simulink model "infinity_mobile_manipulator"  (R2025b)
settings: Solver=ode23t  StartTime=0.0  StopTime=30.0  MaxStep=0.01  RelTol=1e-3  AbsTol=1e-3  EnableMultiTasking=on
undefined symbols (not defined in the file): A, armP, goal, lemP, qa, qb, qHome, Ta, X, Y, Z
libraries: sm_lib x60, nesl_utility x12
(part 2 of 2)

== matlab function infinity_mobile_manipulator/gate ==
  data: v input; w input; vo output; phase input; wo output
function [vo, wo] = gate(v, w, phase)
% Drive only during Navigate/Settle (phase 0); stand still afterwards
if phase == 0
    vo = v; wo = w;
else
    vo = 0; wo = 0;
end

== matlab function infinity_mobile_manipulator/go to goal ==
  data: x input; y input; v output; th input; goal input; w output; reached output
function [v, w, reached] = goToGoal(x, y, th, goal)
kv = 0.6; kw = 2.0; tol = 0.03; vmax = 0.7; wmax = 1.5;   % vmax = QBot nominal speed
dx = goal(1) - x;  dy = goal(2) - y;
rho   = hypot(dx, dy);
ang   = atan2(dy, dx);
alpha = atan2(sin(ang - th), cos(ang - th));              % heading error, wrapped
reached = rho < tol;
if reached
    v = 0; w = 0;
else
    v = min(kv*rho*max(cos(alpha), 0), vmax);
    w = max(min(kw*alpha, wmax), -wmax);
end
end

== stateflow chart infinity_mobile_manipulator/Superviser ==
  settings: updateMethod=DISCRETE  sampleTime=0.01
  state Navigate
    entry:
    phase=0;
    tEnter = tClk;
  state Settle
    entry:
    phase = 0;
    tEnter = tClk;
  state Approach
    entry:
    phase = 1;
    tEnter = tClk;
  state Trace
    entry:
    phase = 2;
    tEnter = tClk;
  (default) -> Navigate
  Navigate -> Settle : [reached]
  Settle -> Approach : [tClk - tEnter >= 1]
  Approach -> Trace : [tClk - tEnter >= 4]
  data: tEnter output double; reached input; phase output double; tClk input double

== matlab function infinity_mobile_manipulator/armRef ==
  data: phase input; qref output; t input; tEnter input; armP input; lemP input; qHome input; Ta input; pd output
function [qref, pd] = armRef(phase, t, tEnter, armP, lemP, qHome, Ta)
qh = qHome(:);
tp = max(t - tEnter, 0);
pStart = lemniscate(0, lemP);
if phase == 1                               % Approach: stowed -> start of the infinity
    u = min(tp/Ta, 1);  s = 3*u^2 - 2*u^3;  % smoothstep
    qref = (1-s)*qh + s*ik4(pStart, armP);
    pd = pStart;
elseif phase == 2                           % Trace: repeats forever
    pd = lemniscate(tp, lemP);
    qref = ik4(pd, armP);
else                                        % Navigate / Settle: stowed
    qref = qh;  pd = pStart;
end
end

function p = lemniscate(t, P)               % P = [cx cy a z w]
d = 1 + sin(P(5)*t)^2;
p = [P(1) + P(3)*cos(P(5)*t)/d;
     P(2) + P(3)*sin(P(5)*t)*cos(P(5)*t)/d;
     P(4)];
end

function q = ik4(p, A)                      % A = [h1 L2 L3 L4], gripper pointing down
h1 = A(1); L2 = A(2); L3 = A(3); L4 = A(4);
q1 = atan2(p(2), p(1));
dr = hypot(p(1), p(2));
dz = p(3) + L4 - h1;
c3 = (dr^2 + dz^2 - L2^2 - L3^2) / (2*L2*L3);
c3 = max(min(c3, 1), -1);
q3 = -acos(c3);                             % elbow up
q2 = atan2(dz, dr) - atan2(L3*sin(q3), L2 + L3*c3);
q4 = -pi/2 - q2 - q3;                       % keeps the gripper vertical
q  = [q1; q2; q3; q4];
end
